simulink model "CRG_Hockenheim_f_preview"  (R2025a)
settings: Solver=VariableStepAuto  StartTime=0.0  StopTime=10.0  RelTol=1e-3  EnableMultiTasking=on
PreLoadFcn:
  | sm_car_scene_stl_create(Scene.CRG_Hockenheim_F)
model workspace (MATLAB code in the model file):
  | load CRG_Custom_f_dat
  | load CRG_Custom_f_trajectory_default
undefined symbols (not defined in the file or in its folder): MDatabase, Scene, X, Y, Z
libraries: sm_lib x6, sm_car_scene_crg_hockenheim_f x1, nesl_utility x1
Description:
  | Copyright 2021-2026 The MathWorks, Inc.
settings Model: Creator=smiller  LastModifiedBy=smiller
settings SolverCC: AlgebraicLoopSolver=TrustRegion
settings DataIOCC: LimitDataPoints=on  ReturnWorkspaceOutputs=off
settings OptimizationCC: ReuseModelBlockBuffer=off  LifeSpan=inf
settings DebuggingCC: UnconnectedInputMsg=warning  UnconnectedOutputMsg=warning  UnconnectedLineMsg=warning  AllowSymbolicDim=off  SFUnexpectedBacktrackingDiag=warning  SFNoUnconditionalDefaultTransitionDiag=warning  SFExecutionAtInitializationDiag=none  ArithmeticOperatorsInVariantConditions=warning
settings ModelReferenceCC: EnableRefExpFcnMdlSchedulingChecks=on
settings SFSimCC: SimUseLocalCustomCode=off  CustomCodeUndefinedFunction=UseInterfaceOnly
settings RTWCC: RTWUseLocalCustomCode=off  GPUComputeCapability=3.5  DLArmComputeVersion=19.05
settings CodeAppCC: StateflowObjectComments=on
settings GRTTargetCC: TargetLangStandard=C89/C90 (ANSI)
settings ConfigComp: CovMetricSettings=dw  CovSaveCumulativeToWorkspaceVar=on  CovSaveSingleToWorkspaceVar=on  CovExternalEMLEnable=off  CovSFcnEnable=off
settings SimscapeCC: SimscapeNominalValues="[{\"value\":\"10\",\"unit\":\"V\"},{\"value\":\"1\",\"unit\":\"A\"},{\"value\":\"10\",\"unit\":\"N*m\"},{\"value\":\"10\",\"unit\":\"bar\"},{\"value\":\"100\",\"unit\":\"kJ/kg\"},{\"value\":\"1\",\"unit\":\"kW\"},{\"value\":\"300\",\"unit\":\"K\"},{\"value\":\"100\",\"unit\":\"cm^3/s\"},{\"value\":\"1\",\"unit\":\"kN\"},{\"value\":\"1\",\"unit\":\"g/cm^3\"},{\"value\":\"1\",\"unit\":\"l\"},{\"value\":\"1\",\"unit\":\"cm^2\"},{\"value\":\"60\",\"unit\":\"Hz\"}]"  SimscapeLogType=all  SimscapeLogDataHistory=10000.0
settings ConfigurationSet: Description=SimMechanics 2G
settings ExplorerConfigSet: InternalSimMechanicsExplorerSettings="<ExplorerConfiguration><canonicalview>default</canonicalview><AnimationSetting><BasePlaybackSpeed>1.0</BasePlaybackSpeed><PlaybackSpeedFactor>1.0</PlaybackSpeedFactor></AnimationSetting><TilePanel><TileInfo><Tiles Columns=\"1\" Count=\"1\" Rows=\"1\"><Column Weight=\"1\"/><Row Weight=\"1\"/><Tile Height=\"1\" Width=\"1\" X=\"0\" Y=\"0\"/></Tiles></TileInfo><SceneInfo><SceneViewer><BGColor><R>1</R><G>1</G><B>1</B></BGColor><Camera><DoPerspective>off</DoPerspective><Position><X>-56.653885984533801</X><Y>-43.5984972402080047</Y><Z>473.161405602841796</Z></Position><Center><X>-56.653885984533801</X><Y>-43.5984972402080047</Y><Z>15.2925731081552385</Z></Center><Up><X>0</X><Y>1</Y><Z>-0</Z></Up><ViewLimDist>1</ViewLimDist><YLim>274.338494567871123</YLim><XLim>425.155737310208337</XLim></Camera></SceneViewer></SceneInfo></TilePanel><MechEditorPanel><Cameras/><GfxPanelCameraMap/><VideoCreator><PlaybackSpeedRatio>1.0</PlaybackSpeedRatio><FrameRate>30</FrameRate><VideoFormat>Motion JPEG AVI</VideoFormat><FrameSize>auto</FrameSize></VideoCreator></MechEditorPanel></ExplorerConfiguration>"

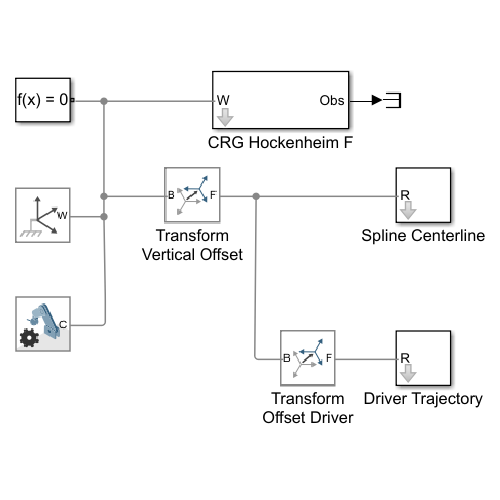
[thumbnail: Simulink's stored preview of the top-level diagram]
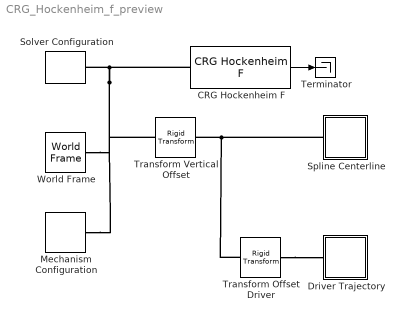
== system CRG_Hockenheim_f_preview ==
  CRG Hockenheim F : sm_car_scene_crg_hockenheim_f/CRG Hockenheim F  geometry=Scene.CRG_Hockenheim_F.Geometry
  Driver Trajectory : Subsystem  mask{driver_traj=MDatabase.CRG_Hockenheim_F.Sedan_Hamba}
      mask prompts: driver_traj "Driver Trajectorz"
  Mechanism Configuration : sm_lib/Utilities/Mechanism Configuration  UniformGravity=Constant  GravityVector=[0 0 -9.80665]  GravityVectorUnits=m/s^2  LinearizationDelta=0.001  JointModeTransitionNonlinearIterations=2
  Solver Configuration : nesl_utility/Solver Configuration  PhysicalDomain=network_engine_domain  SubClassName=solver  LeftPortType=input  RightPortType=generic  Tones=[]  Harmonics=[]  SimulateNoise=off  Profile=off  UseLocalSampling=off  EnableSwitchedLinearOptims=on  FrequencyDomain=off  UseCCode=off  RelTol=0.001  AbsTol=1e-06  MinStep=1e-09  ToWorkspace=off  RevertToSquareIcSolve=off  NumHomotopyIterations=100  PhasorMode=off  PhasorModeNumHarmonics=1  ConsistencySolver=NEWTON_FTOL  IndexReductionMethod=DerivativeReplacement  DoDC=off  ResidualTolerance=1e-09  ConsistencyTolSource=GLOBAL  ConsistencyAbsTol=0.001  ConsistencyRelTol=0.001  ConsistencyTolFactor=0.001  UseLocalSolver=off  LocalSolverChoice=NE_BACKWARD_EULER_ADVANCER  ResolveIndetEquations=on  FunctionEvalNumThread=1  LocalSolverSampleTime=0.001  DoFixedCost=off  MaxNonlinIter=3  MaxModeIter=2  ComputeImpulses=off  ImpulseIterations=2  LinearAlgebra=Sparse  LinearAlgebraNumThread=0  EquationFormulation=NE_TIME_EF  DelaysMemoryBudget=1024  AutomaticFiltering=on  FilteringTimeConstant=0.001  PartitionStorageMethod=AS_NEEDED  PartitionMemoryBudget=1024  PartitionMethod=FAST  MultibodyUseLocalSolver=off  MultibodyLocalSolverChoice=ODE1  MultibodyLocalSolverSampleTime=0.001
  Spline Centerline : Subsystem  mask{centerline=Scene.CRG_Hockenheim_F.Geometry.centerline}
      mask prompts: centerline "Centerline Data"
  Terminator : Terminator
  Transform Offset Driver : sm_lib/Frames and Transforms/Rigid Transform  RotationMethod=None  FollAlignAxisA=+X  BaseAlignAxisA=+Y  FollAlignAxisB=+Y  BaseAlignAxisB=+Z  RotationStandardAxis=+Z  RotationAngle=0.0  RotationAngleUnits=deg  RotationArbitraryAxis=[0 0 1]  RotationSequenceAxes=FollowerAxes  RotationSequence=XYX  RotationSequenceAngles=[0 0 0]  RotationSequenceAnglesUnits=deg  RotationMatrix=[1 0 0; 0 1 0; 0 0 1]  Quaternion=[1 0 0 0]  TranslationMethod=Cartesian  TranslationCartesianOffset=[0 0 0.2]  TranslationCartesianOffsetUnits=m  TranslationStandardAxis=+Z  TranslationStandardOffset=0  TranslationStandardOffsetUnits=m  TranslationROffset=0  TranslationROffsetUnits=m  TranslationThetaOffset=0  TranslationThetaOffsetUnits=deg  TranslationZOffset=0  TranslationZOffsetUnits=m
  Transform Vertical Offset : sm_lib/Frames and Transforms/Rigid Transform  RotationMethod=None  FollAlignAxisA=+X  BaseAlignAxisA=+Y  FollAlignAxisB=+Y  BaseAlignAxisB=+Z  RotationStandardAxis=+Z  RotationAngle=0.0  RotationAngleUnits=deg  RotationArbitraryAxis=[0 0 1]  RotationSequenceAxes=FollowerAxes  RotationSequence=XYX  RotationSequenceAngles=[0 0 0]  RotationSequenceAnglesUnits=deg  RotationMatrix=[1 0 0; 0 1 0; 0 0 1]  Quaternion=[1 0 0 0]  TranslationMethod=Cartesian  TranslationCartesianOffset=[0 0 0.1]  TranslationCartesianOffsetUnits=m  TranslationStandardAxis=+Z  TranslationStandardOffset=0  TranslationStandardOffsetUnits=m  TranslationROffset=0  TranslationROffsetUnits=m  TranslationThetaOffset=0  TranslationThetaOffsetUnits=deg  TranslationZOffset=0  TranslationZOffsetUnits=m
  World Frame : sm_lib/Frames and Transforms/World Frame
  wires:
  CRG Hockenheim F/1 -> Terminator/1
  connections:
  Transform Vertical Offset/LConn1 -- Mechanism Configuration/RConn1 -- World Frame/RConn1 -- CRG Hockenheim F/LConn1 -- Solver Configuration/RConn1
  Transform Offset Driver/LConn1 -- Spline Centerline/LConn1 -- Transform Vertical Offset/RConn1
  Transform Offset Driver/RConn1 -- Driver Trajectory/LConn1

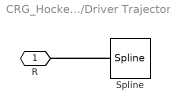
== system CRG_Hockenheim_f_preview/Driver Trajectory ==
  Spline : sm_lib/Curves and Surfaces/Spline  DataPoints=[driver_traj.Trajectory.x.Value' driver_traj.Trajectory.y.Value' driver_traj.Trajectory.z.Value']  DataPointsUnits=m  EndConditionType=Natural  GraphicType=FromGeometry  MarkerShape=Sphere  MarkerSize=10  GraphicVisPropType=SimpleVisualProperties  GraphicDiffuseColor=[0.2 0.6 1.0]  GraphicOpacity=1.0  GraphicSpecularColor=[0.5 0.5 0.5 1.0]  GraphicAmbientColor=[0.15 0.15 0.15 1.0]  GraphicEmissiveColor=[0.0 0.0 0.0 1.0]  GraphicShininess=75
  R : PMIOPort  Side=Left
  connections:
  Spline/LConn1 -- R/RConn1

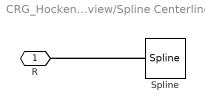
== system CRG_Hockenheim_f_preview/Spline Centerline ==
  Spline : sm_lib/Curves and Surfaces/Spline  DataPoints=centerline.xyz  DataPointsUnits=m  EndConditionType=Natural  GraphicType=FromGeometry  MarkerShape=Sphere  MarkerSize=10  GraphicVisPropType=SimpleVisualProperties  GraphicDiffuseColor=[1.0 0.0 0.2]  GraphicOpacity=1.0  GraphicSpecularColor=[0.5 0.5 0.5 1.0]  GraphicAmbientColor=[0.15 0.15 0.15 1.0]  GraphicEmissiveColor=[0.0 0.0 0.0 1.0]  GraphicShininess=75
  R : PMIOPort  Side=Left
  connections:
  Spline/LConn1 -- R/RConn1
